simulink model "s_c_nbe_m32k"  (R2018a)
settings: Solver=VariableStepDiscrete  StartTime=0.0  StopTime=1000  RelTol=1e-3
undefined symbols (not defined in the file): fft_stages, n_taps, output_bits, pfb_coeff_gen_calc, xengbits
libraries: xbsIndex_r4 x23714, casper_library_misc x17, xps_library x4, casper_library_scopes x4, xbsReplacements_r4 x4
(part 155 of 171)

== system s_c_nbe_m32k/nb_pfb/pfb_fir_generic2/pfb_fir_taps/bus_adder_tree/add_tree1 ==
  sync : Inport
  din1 : Inport  Port=2
  din2 : Inport  Port=3
  din3 : Inport  Port=4
  din4 : Inport  Port=5
  addr1 : xbsIndex_r4/AddSub  mode=Addition  use_carryin=off  use_carryout=off  en=off  latency=7  precision=Full  arith_type=Unsigned  n_bits=16  bin_pt=14  quantization=Truncate  overflow=Wrap  use_behavioral_HDL=on  hw_selection=Fabric  pipelined=on  use_rpm=on  dbl_ovrd=off  block_type=addsub
  addr2 : xbsIndex_r4/AddSub  mode=Addition  use_carryin=off  use_carryout=off  en=off  latency=7  precision=Full  arith_type=Unsigned  n_bits=16  bin_pt=14  quantization=Truncate  overflow=Wrap  use_behavioral_HDL=on  hw_selection=Fabric  pipelined=on  use_rpm=on  dbl_ovrd=off  block_type=addsub
  addr3 : xbsIndex_r4/AddSub  mode=Addition  use_carryin=off  use_carryout=off  en=off  latency=7  precision=Full  arith_type=Unsigned  n_bits=16  bin_pt=14  quantization=Truncate  overflow=Wrap  use_behavioral_HDL=on  hw_selection=Fabric  pipelined=on  use_rpm=on  dbl_ovrd=off  block_type=addsub
  sync_delay : xbsIndex_r4/Delay  rst=off  infoeditControl=Selection of Reset will increase slice count due to use of real FFs and instead of SRLs  en=off  latency=14  reg_retiming=on  dbl_ovrd=off  block_type=delay
      settings: block_version=11.4
  sync_out : Outport
  dout : Outport  Port=2
  wires:
  addr3/1 -> dout/1
  addr2/1 -> addr3/2
  addr1/1 -> addr3/1
  din4/1 -> addr2/2
  din3/1 -> addr2/1
  din2/1 -> addr1/2
  din1/1 -> addr1/1
  sync_delay/1 -> sync_out/1
  sync/1 -> sync_delay/1

== system s_c_nbe_m32k/nb_pfb/pfb_fir_generic2/pfb_fir_taps/bus_adder_tree/d_bussify ==
  in1 : Inport
  in2 : Inport  Port=2
  concatenate : xbsIndex_r4/Concat  num_inputs=2  dbl_ovrd=off  block_type=concat
  reinterpret1 : xbsIndex_r4/Reinterpret  force_arith_type=on  arith_type=Unsigned  force_bin_pt=on  bin_pt=0  block_type=reinterpret
      settings: infoedit="Changes signal type without altering the binary representation.   You can changed the signal between signed and unsigned, and relocate the binary point.<br><br>Hardware notes: In hardware this block costs nothing.<br><br>Example:  Suppose the input is 6 bits wide, signed, with 2 fractional bits, and the output is forced to unsigned with 0 fractional bits.  Then an input of -2.0 (1110.00 in binary 2's complement) becomes an output of 56 (111000 in binary)."
  reinterpret2 : xbsIndex_r4/Reinterpret  force_arith_type=on  arith_type=Unsigned  force_bin_pt=on  bin_pt=0  block_type=reinterpret
      settings: infoedit="Changes signal type without altering the binary representation.   You can changed the signal between signed and unsigned, and relocate the binary point.<br><br>Hardware notes: In hardware this block costs nothing.<br><br>Example:  Suppose the input is 6 bits wide, signed, with 2 fractional bits, and the output is forced to unsigned with 0 fractional bits.  Then an input of -2.0 (1110.00 in binary 2's complement) becomes an output of 56 (111000 in binary)."
  bus_out : Outport
  wires:
  reinterpret2/1 -> concatenate/2
  in2/1 -> reinterpret2/1
  reinterpret1/1 -> concatenate/1
  in1/1 -> reinterpret1/1
  concatenate/1 -> bus_out/1

== system s_c_nbe_m32k/nb_pfb/pfb_fir_generic2/pfb_fir_taps/bus_adder_tree/expand0 ==
  bus_in : Inport
  reinterpret1 : xbsIndex_r4/Reinterpret  force_arith_type=on  arith_type="Signed  (2's comp)"  force_bin_pt=on  bin_pt=34  block_type=reinterpret
  reinterpret2 : xbsIndex_r4/Reinterpret  force_arith_type=on  arith_type="Signed  (2's comp)"  force_bin_pt=on  bin_pt=34  block_type=reinterpret
  slice1 : xbsIndex_r4/Slice  nbits=36  boolean_output=off  mode=Upper Bit Location + Width  bit1=-36  base1=MSB of Input  bit0=0  base0=LSB of Input  dbl_ovrd=off  block_type=slice
  slice2 : xbsIndex_r4/Slice  nbits=36  boolean_output=off  mode=Upper Bit Location + Width  bit1=0  base1=MSB of Input  bit0=0  base0=LSB of Input  dbl_ovrd=off  block_type=slice
  msb_out2 : Outport
  lsb_out1 : Outport  Port=2
  wires:
  bus_in/1 -> slice2/1, slice1/1
  slice2/1 -> reinterpret2/1
  reinterpret2/1 -> msb_out2/1
  slice1/1 -> reinterpret1/1
  reinterpret1/1 -> lsb_out1/1

== system s_c_nbe_m32k/nb_pfb/pfb_fir_generic2/pfb_fir_taps/bus_adder_tree/expand1 ==
  bus_in : Inport
  reinterpret1 : xbsIndex_r4/Reinterpret  force_arith_type=on  arith_type="Signed  (2's comp)"  force_bin_pt=on  bin_pt=34  block_type=reinterpret
  reinterpret2 : xbsIndex_r4/Reinterpret  force_arith_type=on  arith_type="Signed  (2's comp)"  force_bin_pt=on  bin_pt=34  block_type=reinterpret
  slice1 : xbsIndex_r4/Slice  nbits=36  boolean_output=off  mode=Upper Bit Location + Width  bit1=-36  base1=MSB of Input  bit0=0  base0=LSB of Input  dbl_ovrd=off  block_type=slice
  slice2 : xbsIndex_r4/Slice  nbits=36  boolean_output=off  mode=Upper Bit Location + Width  bit1=0  base1=MSB of Input  bit0=0  base0=LSB of Input  dbl_ovrd=off  block_type=slice
  msb_out2 : Outport
  lsb_out1 : Outport  Port=2
  wires:
  bus_in/1 -> slice2/1, slice1/1
  slice2/1 -> reinterpret2/1
  reinterpret2/1 -> msb_out2/1
  slice1/1 -> reinterpret1/1
  reinterpret1/1 -> lsb_out1/1

== system s_c_nbe_m32k/nb_pfb/pfb_fir_generic2/pfb_fir_taps/bus_adder_tree/expand2 ==
  bus_in : Inport
  reinterpret1 : xbsIndex_r4/Reinterpret  force_arith_type=on  arith_type="Signed  (2's comp)"  force_bin_pt=on  bin_pt=34  block_type=reinterpret
  reinterpret2 : xbsIndex_r4/Reinterpret  force_arith_type=on  arith_type="Signed  (2's comp)"  force_bin_pt=on  bin_pt=34  block_type=reinterpret
  slice1 : xbsIndex_r4/Slice  nbits=36  boolean_output=off  mode=Upper Bit Location + Width  bit1=-36  base1=MSB of Input  bit0=0  base0=LSB of Input  dbl_ovrd=off  block_type=slice
  slice2 : xbsIndex_r4/Slice  nbits=36  boolean_output=off  mode=Upper Bit Location + Width  bit1=0  base1=MSB of Input  bit0=0  base0=LSB of Input  dbl_ovrd=off  block_type=slice
  msb_out2 : Outport
  lsb_out1 : Outport  Port=2
  wires:
  bus_in/1 -> slice2/1, slice1/1
  slice2/1 -> reinterpret2/1
  reinterpret2/1 -> msb_out2/1
  slice1/1 -> reinterpret1/1
  reinterpret1/1 -> lsb_out1/1

== system s_c_nbe_m32k/nb_pfb/pfb_fir_generic2/pfb_fir_taps/bus_adder_tree/expand3 ==
  bus_in : Inport
  reinterpret1 : xbsIndex_r4/Reinterpret  force_arith_type=on  arith_type="Signed  (2's comp)"  force_bin_pt=on  bin_pt=34  block_type=reinterpret
  reinterpret2 : xbsIndex_r4/Reinterpret  force_arith_type=on  arith_type="Signed  (2's comp)"  force_bin_pt=on  bin_pt=34  block_type=reinterpret
  slice1 : xbsIndex_r4/Slice  nbits=36  boolean_output=off  mode=Upper Bit Location + Width  bit1=-36  base1=MSB of Input  bit0=0  base0=LSB of Input  dbl_ovrd=off  block_type=slice
  slice2 : xbsIndex_r4/Slice  nbits=36  boolean_output=off  mode=Upper Bit Location + Width  bit1=0  base1=MSB of Input  bit0=0  base0=LSB of Input  dbl_ovrd=off  block_type=slice
  msb_out2 : Outport
  lsb_out1 : Outport  Port=2
  wires:
  bus_in/1 -> slice2/1, slice1/1
  slice2/1 -> reinterpret2/1
  reinterpret2/1 -> msb_out2/1
  slice1/1 -> reinterpret1/1
  reinterpret1/1 -> lsb_out1/1

== system s_c_nbe_m32k/nb_pfb/pfb_fir_generic2/pfb_fir_taps/bus_mult/a*b_bussify ==
  in1 : Inport
  in2 : Inport  Port=2
  in3 : Inport  Port=3
  in4 : Inport  Port=4
  in5 : Inport  Port=5
  in6 : Inport  Port=6
  in7 : Inport  Port=7
  in8 : Inport  Port=8
  concatenate : xbsIndex_r4/Concat  num_inputs=8  dbl_ovrd=off  block_type=concat
  reinterpret{1..8} (8 alike) : xbsIndex_r4/Reinterpret  force_arith_type=on  arith_type=Unsigned  force_bin_pt=on  bin_pt=0  block_type=reinterpret
      reinterpret1 settings: infoedit="Changes signal type without altering the binary representation.   You can changed the signal between signed and unsigned, and relocate the binary point.<br><br>Hardware notes: In hardware this block costs nothing.<br><br>Example:  Suppose the input is 6 bits wide, signed, with 2 fractional bits, and the output is forced to unsigned with 0 fractional bits.  Then an input of -2.0 (1110.00 in binary 2's complement) becomes an output of 56 (111000 in binary)."
      reinterpret2 settings: infoedit="Changes signal type without altering the binary representation.   You can changed the signal between signed and unsigned, and relocate the binary point.<br><br>Hardware notes: In hardware this block costs nothing.<br><br>Example:  Suppose the input is 6 bits wide, signed, with 2 fractional bits, and the output is forced to unsigned with 0 fractional bits.  Then an input of -2.0 (1110.00 in binary 2's complement) becomes an output of 56 (111000 in binary)."
  bus_out : Outport
  wires:
  reinterpret8/1 -> concatenate/8
  in8/1 -> reinterpret8/1
  reinterpret7/1 -> concatenate/7
  in7/1 -> reinterpret7/1
  reinterpret6/1 -> concatenate/6
  in6/1 -> reinterpret6/1
  reinterpret5/1 -> concatenate/5
  in5/1 -> reinterpret5/1
  reinterpret4/1 -> concatenate/4
  in4/1 -> reinterpret4/1
  reinterpret3/1 -> concatenate/3
  in3/1 -> reinterpret3/1
  reinterpret2/1 -> concatenate/2
  in2/1 -> reinterpret2/1
  reinterpret1/1 -> concatenate/1
  in1/1 -> reinterpret1/1
  concatenate/1 -> bus_out/1

== system s_c_nbe_m32k/nb_pfb/pfb_fir_generic2/pfb_fir_taps/bus_mult/a_debus ==
  bus_in : Inport
  reinterpret{1..8} (8 alike) : xbsIndex_r4/Reinterpret  force_arith_type=on  arith_type="Signed  (2's comp)"  force_bin_pt=on  bin_pt=17  block_type=reinterpret
  slice1 : xbsIndex_r4/Slice  nbits=18  boolean_output=off  mode=Upper Bit Location + Width  bit1=-126  base1=MSB of Input  bit0=0  base0=LSB of Input  dbl_ovrd=off  block_type=slice
  slice2 : xbsIndex_r4/Slice  nbits=18  boolean_output=off  mode=Upper Bit Location + Width  bit1=-108  base1=MSB of Input  bit0=0  base0=LSB of Input  dbl_ovrd=off  block_type=slice
  slice3 : xbsIndex_r4/Slice  nbits=18  boolean_output=off  mode=Upper Bit Location + Width  bit1=-90  base1=MSB of Input  bit0=0  base0=LSB of Input  dbl_ovrd=off  block_type=slice
  slice4 : xbsIndex_r4/Slice  nbits=18  boolean_output=off  mode=Upper Bit Location + Width  bit1=-72  base1=MSB of Input  bit0=0  base0=LSB of Input  dbl_ovrd=off  block_type=slice
  slice5 : xbsIndex_r4/Slice  nbits=18  boolean_output=off  mode=Upper Bit Location + Width  bit1=-54  base1=MSB of Input  bit0=0  base0=LSB of Input  dbl_ovrd=off  block_type=slice
  slice6 : xbsIndex_r4/Slice  nbits=18  boolean_output=off  mode=Upper Bit Location + Width  bit1=-36  base1=MSB of Input  bit0=0  base0=LSB of Input  dbl_ovrd=off  block_type=slice
  slice7 : xbsIndex_r4/Slice  nbits=18  boolean_output=off  mode=Upper Bit Location + Width  bit1=-18  base1=MSB of Input  bit0=0  base0=LSB of Input  dbl_ovrd=off  block_type=slice
  slice8 : xbsIndex_r4/Slice  nbits=18  boolean_output=off  mode=Upper Bit Location + Width  bit1=0  base1=MSB of Input  bit0=0  base0=LSB of Input  dbl_ovrd=off  block_type=slice
  msb_out8 : Outport
  out7 : Outport  Port=2
  out6 : Outport  Port=3
  out5 : Outport  Port=4
  out4 : Outport  Port=5
  out3 : Outport  Port=6
  out2 : Outport  Port=7
  lsb_out1 : Outport  Port=8
  wires:
  bus_in/1 -> slice8/1, slice7/1, slice6/1, slice5/1, slice4/1, slice3/1, slice2/1, slice1/1
  slice8/1 -> reinterpret8/1
  reinterpret8/1 -> msb_out8/1
  slice7/1 -> reinterpret7/1
  reinterpret7/1 -> out7/1
  slice6/1 -> reinterpret6/1
  reinterpret6/1 -> out6/1
  slice5/1 -> reinterpret5/1
  reinterpret5/1 -> out5/1
  slice4/1 -> reinterpret4/1
  reinterpret4/1 -> out4/1
  slice3/1 -> reinterpret3/1
  reinterpret3/1 -> out3/1
  slice2/1 -> reinterpret2/1
  reinterpret2/1 -> out2/1
  slice1/1 -> reinterpret1/1
  reinterpret1/1 -> lsb_out1/1

== system s_c_nbe_m32k/nb_pfb/pfb_fir_generic2/pfb_fir_taps/bus_mult/b_debus ==
  bus_in : Inport
  reinterpret{1..8} (8 alike) : xbsIndex_r4/Reinterpret  force_arith_type=on  arith_type="Signed  (2's comp)"  force_bin_pt=on  bin_pt=17  block_type=reinterpret
  slice1 : xbsIndex_r4/Slice  nbits=18  boolean_output=off  mode=Upper Bit Location + Width  bit1=-126  base1=MSB of Input  bit0=0  base0=LSB of Input  dbl_ovrd=off  block_type=slice
  slice2 : xbsIndex_r4/Slice  nbits=18  boolean_output=off  mode=Upper Bit Location + Width  bit1=-108  base1=MSB of Input  bit0=0  base0=LSB of Input  dbl_ovrd=off  block_type=slice
  slice3 : xbsIndex_r4/Slice  nbits=18  boolean_output=off  mode=Upper Bit Location + Width  bit1=-90  base1=MSB of Input  bit0=0  base0=LSB of Input  dbl_ovrd=off  block_type=slice
  slice4 : xbsIndex_r4/Slice  nbits=18  boolean_output=off  mode=Upper Bit Location + Width  bit1=-72  base1=MSB of Input  bit0=0  base0=LSB of Input  dbl_ovrd=off  block_type=slice
  slice5 : xbsIndex_r4/Slice  nbits=18  boolean_output=off  mode=Upper Bit Location + Width  bit1=-54  base1=MSB of Input  bit0=0  base0=LSB of Input  dbl_ovrd=off  block_type=slice
  slice6 : xbsIndex_r4/Slice  nbits=18  boolean_output=off  mode=Upper Bit Location + Width  bit1=-36  base1=MSB of Input  bit0=0  base0=LSB of Input  dbl_ovrd=off  block_type=slice
  slice7 : xbsIndex_r4/Slice  nbits=18  boolean_output=off  mode=Upper Bit Location + Width  bit1=-18  base1=MSB of Input  bit0=0  base0=LSB of Input  dbl_ovrd=off  block_type=slice
  slice8 : xbsIndex_r4/Slice  nbits=18  boolean_output=off  mode=Upper Bit Location + Width  bit1=0  base1=MSB of Input  bit0=0  base0=LSB of Input  dbl_ovrd=off  block_type=slice
  msb_out8 : Outport
  out7 : Outport  Port=2
  out6 : Outport  Port=3
  out5 : Outport  Port=4
  out4 : Outport  Port=5
  out3 : Outport  Port=6
  out2 : Outport  Port=7
  lsb_out1 : Outport  Port=8
  wires:
  bus_in/1 -> slice8/1, slice7/1, slice6/1, slice5/1, slice4/1, slice3/1, slice2/1, slice1/1
  slice8/1 -> reinterpret8/1
  reinterpret8/1 -> msb_out8/1
  slice7/1 -> reinterpret7/1
  reinterpret7/1 -> out7/1
  slice6/1 -> reinterpret6/1
  reinterpret6/1 -> out6/1
  slice5/1 -> reinterpret5/1
  reinterpret5/1 -> out5/1
  slice4/1 -> reinterpret4/1
  reinterpret4/1 -> out4/1
  slice3/1 -> reinterpret3/1
  reinterpret3/1 -> out3/1
  slice2/1 -> reinterpret2/1
  reinterpret2/1 -> out2/1
  slice1/1 -> reinterpret1/1
  reinterpret1/1 -> lsb_out1/1

== system s_c_nbe_m32k/nb_pfb/pfb_fir_generic2/pfb_fir_taps/bus_mult/repa ==
  in : Inport
  bussify : Subsystem  mask(bus_create){inputNum=1}
      mask prompts: inputNum "Number of inputs:"
      mask init:
      | bus_create_init(gcb,...
      |     'inputNum', inputNum);
  out : Outport
  wires:
  bussify/1(bus_out) -> out/1
  in/1 -> bussify/1(in1)

== system s_c_nbe_m32k/nb_pfb/pfb_fir_generic2/pfb_fir_taps/bus_mult/repb ==
  in : Inport
  bussify : Subsystem  mask(bus_create){inputNum=1}
      mask prompts: inputNum "Number of inputs:"
      mask init:
      | bus_create_init(gcb,...
      |     'inputNum', inputNum);
  out : Outport
  wires:
  bussify/1(bus_out) -> out/1
  in/1 -> bussify/1(in1)

== system s_c_nbe_m32k/nb_pfb/pfb_fir_generic2/pfb_fir_taps/tap_delays/A_bussify0 ==
  in1 : Inport
  in2 : Inport  Port=2
  in3 : Inport  Port=3
  in4 : Inport  Port=4
  in5 : Inport  Port=5
  in6 : Inport  Port=6
  in7 : Inport  Port=7
  in8 : Inport  Port=8
  in9 : Inport  Port=9
  in10 : Inport  Port=10
  in11 : Inport  Port=11
  in12 : Inport  Port=12
  in13 : Inport  Port=13
  in14 : Inport  Port=14
  in15 : Inport  Port=15
  in16 : Inport  Port=16
  in17 : Inport  Port=17
  in18 : Inport  Port=18
  in19 : Inport  Port=19
  in20 : Inport  Port=20
  in21 : Inport  Port=21
  in22 : Inport  Port=22
  in23 : Inport  Port=23
  in24 : Inport  Port=24
  in25 : Inport  Port=25
  in26 : Inport  Port=26
  in27 : Inport  Port=27
  in28 : Inport  Port=28
  in29 : Inport  Port=29
  in30 : Inport  Port=30
  in31 : Inport  Port=31
  in32 : Inport  Port=32
  in33 : Inport  Port=33
  in34 : Inport  Port=34
  in35 : Inport  Port=35
  in36 : Inport  Port=36
  in37 : Inport  Port=37
  in38 : Inport  Port=38
  in39 : Inport  Port=39
  in40 : Inport  Port=40
  in41 : Inport  Port=41
  in42 : Inport  Port=42
  in43 : Inport  Port=43
  in44 : Inport  Port=44
  in45 : Inport  Port=45
  in46 : Inport  Port=46
  in47 : Inport  Port=47
  in48 : Inport  Port=48
  in49 : Inport  Port=49
  in50 : Inport  Port=50
  in51 : Inport  Port=51
  in52 : Inport  Port=52
  in53 : Inport  Port=53
  in54 : Inport  Port=54
  in55 : Inport  Port=55
  in56 : Inport  Port=56
  in57 : Inport  Port=57
  in58 : Inport  Port=58
  in59 : Inport  Port=59
  in60 : Inport  Port=60
  in61 : Inport  Port=61
  in62 : Inport  Port=62
  in63 : Inport  Port=63
  in64 : Inport  Port=64
  in65 : Inport  Port=65
  in66 : Inport  Port=66
  in67 : Inport  Port=67
  in68 : Inport  Port=68
  in69 : Inport  Port=69
  in70 : Inport  Port=70
  in71 : Inport  Port=71
  in72 : Inport  Port=72
  in73 : Inport  Port=73
  in74 : Inport  Port=74
  in75 : Inport  Port=75
  in76 : Inport  Port=76
  in77 : Inport  Port=77
  in78 : Inport  Port=78
  in79 : Inport  Port=79
  in80 : Inport  Port=80
  in81 : Inport  Port=81
  in82 : Inport  Port=82
  in83 : Inport  Port=83
  in84 : Inport  Port=84
  in85 : Inport  Port=85
  in86 : Inport  Port=86
  in87 : Inport  Port=87
  in88 : Inport  Port=88
  in89 : Inport  Port=89
  in90 : Inport  Port=90
  in91 : Inport  Port=91
  in92 : Inport  Port=92
  in93 : Inport  Port=93
  in94 : Inport  Port=94
  in95 : Inport  Port=95
  in96 : Inport  Port=96
  in97 : Inport  Port=97
  in98 : Inport  Port=98
  in99 : Inport  Port=99
  in100 : Inport  Port=100
  in101 : Inport  Port=101
  in102 : Inport  Port=102
  in103 : Inport  Port=103
  in104 : Inport  Port=104
  in105 : Inport  Port=105
  in106 : Inport  Port=106
  in107 : Inport  Port=107
  in108 : Inport  Port=108
  concatenate : xbsIndex_r4/Concat  num_inputs=108  dbl_ovrd=off  block_type=concat
  reinterpret{1..108} (108 alike) : xbsIndex_r4/Reinterpret  force_arith_type=on  arith_type=Unsigned  force_bin_pt=on  bin_pt=0  block_type=reinterpret
      reinterpret1 settings: infoedit="Changes signal type without altering the binary representation.   You can changed the signal between signed and unsigned, and relocate the binary point.<br><br>Hardware notes: In hardware this block costs nothing.<br><br>Example:  Suppose the input is 6 bits wide, signed, with 2 fractional bits, and the output is forced to unsigned with 0 fractional bits.  Then an input of -2.0 (1110.00 in binary 2's complement) becomes an output of 56 (111000 in binary)."
      reinterpret2 settings: infoedit="Changes signal type without altering the binary representation.   You can changed the signal between signed and unsigned, and relocate the binary point.<br><br>Hardware notes: In hardware this block costs nothing.<br><br>Example:  Suppose the input is 6 bits wide, signed, with 2 fractional bits, and the output is forced to unsigned with 0 fractional bits.  Then an input of -2.0 (1110.00 in binary 2's complement) becomes an output of 56 (111000 in binary)."
  bus_out : Outport
  wires:
  reinterpret108/1 -> concatenate/108
  in108/1 -> reinterpret108/1
  reinterpret107/1 -> concatenate/107
  in107/1 -> reinterpret107/1
  reinterpret106/1 -> concatenate/106
  in106/1 -> reinterpret106/1
  reinterpret105/1 -> concatenate/105
  in105/1 -> reinterpret105/1
  reinterpret104/1 -> concatenate/104
  in104/1 -> reinterpret104/1
  reinterpret103/1 -> concatenate/103
  in103/1 -> reinterpret103/1
  reinterpret102/1 -> concatenate/102
  in102/1 -> reinterpret102/1
  reinterpret101/1 -> concatenate/101
  in101/1 -> reinterpret101/1
  reinterpret100/1 -> concatenate/100
  in100/1 -> reinterpret100/1
  reinterpret99/1 -> concatenate/99
  in99/1 -> reinterpret99/1
  reinterpret98/1 -> concatenate/98
  in98/1 -> reinterpret98/1
  reinterpret97/1 -> concatenate/97
  in97/1 -> reinterpret97/1
  reinterpret96/1 -> concatenate/96
  in96/1 -> reinterpret96/1
  reinterpret95/1 -> concatenate/95
  in95/1 -> reinterpret95/1
  reinterpret94/1 -> concatenate/94
  in94/1 -> reinterpret94/1
  reinterpret93/1 -> concatenate/93
  in93/1 -> reinterpret93/1
  reinterpret92/1 -> concatenate/92
  in92/1 -> reinterpret92/1
  reinterpret91/1 -> concatenate/91
  in91/1 -> reinterpret91/1
  reinterpret90/1 -> concatenate/90
  in90/1 -> reinterpret90/1
  reinterpret89/1 -> concatenate/89
  in89/1 -> reinterpret89/1
  reinterpret88/1 -> concatenate/88
  in88/1 -> reinterpret88/1
  reinterpret87/1 -> concatenate/87
  in87/1 -> reinterpret87/1
  reinterpret86/1 -> concatenate/86
  in86/1 -> reinterpret86/1
  reinterpret85/1 -> concatenate/85
  in85/1 -> reinterpret85/1
  reinterpret84/1 -> concatenate/84
  in84/1 -> reinterpret84/1
  reinterpret83/1 -> concatenate/83
  in83/1 -> reinterpret83/1
  reinterpret82/1 -> concatenate/82
  in82/1 -> reinterpret82/1
  reinterpret81/1 -> concatenate/81
  in81/1 -> reinterpret81/1
  reinterpret80/1 -> concatenate/80
  in80/1 -> reinterpret80/1
  reinterpret79/1 -> concatenate/79
  in79/1 -> reinterpret79/1
  reinterpret78/1 -> concatenate/78
  in78/1 -> reinterpret78/1
  reinterpret77/1 -> concatenate/77
  in77/1 -> reinterpret77/1
  reinterpret76/1 -> concatenate/76
  in76/1 -> reinterpret76/1
  reinterpret75/1 -> concatenate/75
  in75/1 -> reinterpret75/1
  reinterpret74/1 -> concatenate/74
  in74/1 -> reinterpret74/1
  reinterpret73/1 -> concatenate/73
  in73/1 -> reinterpret73/1
  reinterpret72/1 -> concatenate/72
  in72/1 -> reinterpret72/1
  reinterpret71/1 -> concatenate/71
  in71/1 -> reinterpret71/1
  reinterpret70/1 -> concatenate/70
  in70/1 -> reinterpret70/1
  reinterpret69/1 -> concatenate/69
  in69/1 -> reinterpret69/1
  reinterpret68/1 -> concatenate/68
  in68/1 -> reinterpret68/1
  reinterpret67/1 -> concatenate/67
  in67/1 -> reinterpret67/1
  reinterpret66/1 -> concatenate/66
  in66/1 -> reinterpret66/1
  reinterpret65/1 -> concatenate/65
  in65/1 -> reinterpret65/1
  reinterpret64/1 -> concatenate/64
  in64/1 -> reinterpret64/1
  reinterpret63/1 -> concatenate/63
  in63/1 -> reinterpret63/1
  reinterpret62/1 -> concatenate/62
  in62/1 -> reinterpret62/1
  reinterpret61/1 -> concatenate/61
  in61/1 -> reinterpret61/1
  reinterpret60/1 -> concatenate/60
  in60/1 -> reinterpret60/1
  reinterpret59/1 -> concatenate/59
  in59/1 -> reinterpret59/1
  reinterpret58/1 -> concatenate/58
  in58/1 -> reinterpret58/1
  reinterpret57/1 -> concatenate/57
  in57/1 -> reinterpret57/1
  reinterpret56/1 -> concatenate/56
  in56/1 -> reinterpret56/1
  reinterpret55/1 -> concatenate/55
  in55/1 -> reinterpret55/1
  reinterpret54/1 -> concatenate/54
  in54/1 -> reinterpret54/1
  reinterpret53/1 -> concatenate/53
  in53/1 -> reinterpret53/1
  reinterpret52/1 -> concatenate/52
  in52/1 -> reinterpret52/1
  reinterpret51/1 -> concatenate/51
  in51/1 -> reinterpret51/1
  reinterpret50/1 -> concatenate/50
  in50/1 -> reinterpret50/1
  reinterpret49/1 -> concatenate/49
  in49/1 -> reinterpret49/1
  reinterpret48/1 -> concatenate/48
  in48/1 -> reinterpret48/1
  reinterpret47/1 -> concatenate/47
  in47/1 -> reinterpret47/1
  reinterpret46/1 -> concatenate/46
  in46/1 -> reinterpret46/1
  reinterpret45/1 -> concatenate/45
  in45/1 -> reinterpret45/1
  reinterpret44/1 -> concatenate/44
  in44/1 -> reinterpret44/1
  reinterpret43/1 -> concatenate/43
  in43/1 -> reinterpret43/1
  reinterpret42/1 -> concatenate/42
  in42/1 -> reinterpret42/1
  reinterpret41/1 -> concatenate/41
  in41/1 -> reinterpret41/1
  reinterpret40/1 -> concatenate/40
  in40/1 -> reinterpret40/1
  reinterpret39/1 -> concatenate/39
  in39/1 -> reinterpret39/1
  reinterpret38/1 -> concatenate/38
  in38/1 -> reinterpret38/1
  reinterpret37/1 -> concatenate/37
  in37/1 -> reinterpret37/1
  reinterpret36/1 -> concatenate/36
  in36/1 -> reinterpret36/1
  reinterpret35/1 -> concatenate/35
  in35/1 -> reinterpret35/1
  reinterpret34/1 -> concatenate/34
  in34/1 -> reinterpret34/1
  reinterpret33/1 -> concatenate/33
  in33/1 -> reinterpret33/1
  reinterpret32/1 -> concatenate/32
  in32/1 -> reinterpret32/1
  reinterpret31/1 -> concatenate/31
  in31/1 -> reinterpret31/1
  reinterpret30/1 -> concatenate/30
  in30/1 -> reinterpret30/1
  reinterpret29/1 -> concatenate/29
  in29/1 -> reinterpret29/1
  reinterpret28/1 -> concatenate/28
  in28/1 -> reinterpret28/1
  reinterpret27/1 -> concatenate/27
  in27/1 -> reinterpret27/1
  reinterpret26/1 -> concatenate/26
  in26/1 -> reinterpret26/1
  reinterpret25/1 -> concatenate/25
  in25/1 -> reinterpret25/1
  reinterpret24/1 -> concatenate/24
  in24/1 -> reinterpret24/1
  reinterpret23/1 -> concatenate/23
  in23/1 -> reinterpret23/1
  reinterpret22/1 -> concatenate/22
  in22/1 -> reinterpret22/1
  reinterpret21/1 -> concatenate/21
  in21/1 -> reinterpret21/1
  reinterpret20/1 -> concatenate/20
  in20/1 -> reinterpret20/1
  reinterpret19/1 -> concatenate/19
  in19/1 -> reinterpret19/1
  reinterpret18/1 -> concatenate/18
  in18/1 -> reinterpret18/1
  reinterpret17/1 -> concatenate/17
  in17/1 -> reinterpret17/1
  reinterpret16/1 -> concatenate/16
  in16/1 -> reinterpret16/1
  reinterpret15/1 -> concatenate/15
  in15/1 -> reinterpret15/1
  reinterpret14/1 -> concatenate/14
  in14/1 -> reinterpret14/1
  reinterpret13/1 -> concatenate/13
  in13/1 -> reinterpret13/1
  reinterpret12/1 -> concatenate/12
  in12/1 -> reinterpret12/1
  reinterpret11/1 -> concatenate/11
  in11/1 -> reinterpret11/1
  reinterpret10/1 -> concatenate/10
  in10/1 -> reinterpret10/1
  reinterpret9/1 -> concatenate/9
  in9/1 -> reinterpret9/1
  reinterpret8/1 -> concatenate/8
  in8/1 -> reinterpret8/1
  reinterpret7/1 -> concatenate/7
  in7/1 -> reinterpret7/1
  reinterpret6/1 -> concatenate/6
  in6/1 -> reinterpret6/1
  reinterpret5/1 -> concatenate/5
  in5/1 -> reinterpret5/1
  reinterpret4/1 -> concatenate/4
  in4/1 -> reinterpret4/1
  reinterpret3/1 -> concatenate/3
  in3/1 -> reinterpret3/1
  reinterpret2/1 -> concatenate/2
  in2/1 -> reinterpret2/1
  reinterpret1/1 -> concatenate/1
  in1/1 -> reinterpret1/1
  concatenate/1 -> bus_out/1

== system s_c_nbe_m32k/nb_pfb/pfb_fir_generic2/pfb_fir_taps/tap_delays/B_bussify0 ==
  in1 : Inport
  in2 : Inport  Port=2
  in3 : Inport  Port=3
  in4 : Inport  Port=4
  in5 : Inport  Port=5
  in6 : Inport  Port=6
  in7 : Inport  Port=7
  in8 : Inport  Port=8
  in9 : Inport  Port=9
  in10 : Inport  Port=10
  in11 : Inport  Port=11
  in12 : Inport  Port=12
  in13 : Inport  Port=13
  in14 : Inport  Port=14
  in15 : Inport  Port=15
  in16 : Inport  Port=16
  in17 : Inport  Port=17
  in18 : Inport  Port=18
  in19 : Inport  Port=19
  in20 : Inport  Port=20
  in21 : Inport  Port=21
  in22 : Inport  Port=22
  in23 : Inport  Port=23
  in24 : Inport  Port=24
  in25 : Inport  Port=25
  in26 : Inport  Port=26
  in27 : Inport  Port=27
  in28 : Inport  Port=28
  in29 : Inport  Port=29
  in30 : Inport  Port=30
  in31 : Inport  Port=31
  in32 : Inport  Port=32
  in33 : Inport  Port=33
  in34 : Inport  Port=34
  in35 : Inport  Port=35
  in36 : Inport  Port=36
  in37 : Inport  Port=37
  in38 : Inport  Port=38
  in39 : Inport  Port=39
  in40 : Inport  Port=40
  in41 : Inport  Port=41
  in42 : Inport  Port=42
  in43 : Inport  Port=43
  in44 : Inport  Port=44
  in45 : Inport  Port=45
  in46 : Inport  Port=46
  in47 : Inport  Port=47
  in48 : Inport  Port=48
  in49 : Inport  Port=49
  in50 : Inport  Port=50
  in51 : Inport  Port=51
  in52 : Inport  Port=52
  in53 : Inport  Port=53
  in54 : Inport  Port=54
  in55 : Inport  Port=55
  in56 : Inport  Port=56
  in57 : Inport  Port=57
  in58 : Inport  Port=58
  in59 : Inport  Port=59
  in60 : Inport  Port=60
  in61 : Inport  Port=61
  in62 : Inport  Port=62
  in63 : Inport  Port=63
  in64 : Inport  Port=64
  in65 : Inport  Port=65
  in66 : Inport  Port=66
  in67 : Inport  Port=67
  in68 : Inport  Port=68
  in69 : Inport  Port=69
  in70 : Inport  Port=70
  in71 : Inport  Port=71
  in72 : Inport  Port=72
  in73 : Inport  Port=73
  in74 : Inport  Port=74
  in75 : Inport  Port=75
  in76 : Inport  Port=76
  in77 : Inport  Port=77
  in78 : Inport  Port=78
  in79 : Inport  Port=79
  in80 : Inport  Port=80
  in81 : Inport  Port=81
  in82 : Inport  Port=82
  in83 : Inport  Port=83
  in84 : Inport  Port=84
  in85 : Inport  Port=85
  in86 : Inport  Port=86
  in87 : Inport  Port=87
  in88 : Inport  Port=88
  in89 : Inport  Port=89
  in90 : Inport  Port=90
  in91 : Inport  Port=91
  in92 : Inport  Port=92
  in93 : Inport  Port=93
  in94 : Inport  Port=94
  in95 : Inport  Port=95
  in96 : Inport  Port=96
  in97 : Inport  Port=97
  in98 : Inport  Port=98
  in99 : Inport  Port=99
  in100 : Inport  Port=100
  in101 : Inport  Port=101
  in102 : Inport  Port=102
  in103 : Inport  Port=103
  in104 : Inport  Port=104
  in105 : Inport  Port=105
  in106 : Inport  Port=106
  in107 : Inport  Port=107
  in108 : Inport  Port=108
  concatenate : xbsIndex_r4/Concat  num_inputs=108  dbl_ovrd=off  block_type=concat
  reinterpret{1..108} (108 alike) : xbsIndex_r4/Reinterpret  force_arith_type=on  arith_type=Unsigned  force_bin_pt=on  bin_pt=0  block_type=reinterpret
      reinterpret1 settings: infoedit="Changes signal type without altering the binary representation.   You can changed the signal between signed and unsigned, and relocate the binary point.<br><br>Hardware notes: In hardware this block costs nothing.<br><br>Example:  Suppose the input is 6 bits wide, signed, with 2 fractional bits, and the output is forced to unsigned with 0 fractional bits.  Then an input of -2.0 (1110.00 in binary 2's complement) becomes an output of 56 (111000 in binary)."
      reinterpret2 settings: infoedit="Changes signal type without altering the binary representation.   You can changed the signal between signed and unsigned, and relocate the binary point.<br><br>Hardware notes: In hardware this block costs nothing.<br><br>Example:  Suppose the input is 6 bits wide, signed, with 2 fractional bits, and the output is forced to unsigned with 0 fractional bits.  Then an input of -2.0 (1110.00 in binary 2's complement) becomes an output of 56 (111000 in binary)."
  bus_out : Outport
  wires:
  reinterpret108/1 -> concatenate/108
  in108/1 -> reinterpret108/1
  reinterpret107/1 -> concatenate/107
  in107/1 -> reinterpret107/1
  reinterpret106/1 -> concatenate/106
  in106/1 -> reinterpret106/1
  reinterpret105/1 -> concatenate/105
  in105/1 -> reinterpret105/1
  reinterpret104/1 -> concatenate/104
  in104/1 -> reinterpret104/1
  reinterpret103/1 -> concatenate/103
  in103/1 -> reinterpret103/1
  reinterpret102/1 -> concatenate/102
  in102/1 -> reinterpret102/1
  reinterpret101/1 -> concatenate/101
  in101/1 -> reinterpret101/1
  reinterpret100/1 -> concatenate/100
  in100/1 -> reinterpret100/1
  reinterpret99/1 -> concatenate/99
  in99/1 -> reinterpret99/1
  reinterpret98/1 -> concatenate/98
  in98/1 -> reinterpret98/1
  reinterpret97/1 -> concatenate/97
  in97/1 -> reinterpret97/1
  reinterpret96/1 -> concatenate/96
  in96/1 -> reinterpret96/1
  reinterpret95/1 -> concatenate/95
  in95/1 -> reinterpret95/1
  reinterpret94/1 -> concatenate/94
  in94/1 -> reinterpret94/1
  reinterpret93/1 -> concatenate/93
  in93/1 -> reinterpret93/1
  reinterpret92/1 -> concatenate/92
  in92/1 -> reinterpret92/1
  reinterpret91/1 -> concatenate/91
  in91/1 -> reinterpret91/1
  reinterpret90/1 -> concatenate/90
  in90/1 -> reinterpret90/1
  reinterpret89/1 -> concatenate/89
  in89/1 -> reinterpret89/1
  reinterpret88/1 -> concatenate/88
  in88/1 -> reinterpret88/1
  reinterpret87/1 -> concatenate/87
  in87/1 -> reinterpret87/1
  reinterpret86/1 -> concatenate/86
  in86/1 -> reinterpret86/1
  reinterpret85/1 -> concatenate/85
  in85/1 -> reinterpret85/1
  reinterpret84/1 -> concatenate/84
  in84/1 -> reinterpret84/1
  reinterpret83/1 -> concatenate/83
  in83/1 -> reinterpret83/1
  reinterpret82/1 -> concatenate/82
  in82/1 -> reinterpret82/1
  reinterpret81/1 -> concatenate/81
  in81/1 -> reinterpret81/1
  reinterpret80/1 -> concatenate/80
  in80/1 -> reinterpret80/1
  reinterpret79/1 -> concatenate/79
  in79/1 -> reinterpret79/1
  reinterpret78/1 -> concatenate/78
  in78/1 -> reinterpret78/1
  reinterpret77/1 -> concatenate/77
  in77/1 -> reinterpret77/1
  reinterpret76/1 -> concatenate/76
  in76/1 -> reinterpret76/1
  reinterpret75/1 -> concatenate/75
  in75/1 -> reinterpret75/1
  reinterpret74/1 -> concatenate/74
  in74/1 -> reinterpret74/1
  reinterpret73/1 -> concatenate/73
  in73/1 -> reinterpret73/1
  reinterpret72/1 -> concatenate/72
  in72/1 -> reinterpret72/1
  reinterpret71/1 -> concatenate/71
  in71/1 -> reinterpret71/1
  reinterpret70/1 -> concatenate/70
  in70/1 -> reinterpret70/1
  reinterpret69/1 -> concatenate/69
  in69/1 -> reinterpret69/1
  reinterpret68/1 -> concatenate/68
  in68/1 -> reinterpret68/1
  reinterpret67/1 -> concatenate/67
  in67/1 -> reinterpret67/1
  reinterpret66/1 -> concatenate/66
  in66/1 -> reinterpret66/1
  reinterpret65/1 -> concatenate/65
  in65/1 -> reinterpret65/1
  reinterpret64/1 -> concatenate/64
  in64/1 -> reinterpret64/1
  reinterpret63/1 -> concatenate/63
  in63/1 -> reinterpret63/1
  reinterpret62/1 -> concatenate/62
  in62/1 -> reinterpret62/1
  reinterpret61/1 -> concatenate/61
  in61/1 -> reinterpret61/1
  reinterpret60/1 -> concatenate/60
  in60/1 -> reinterpret60/1
  reinterpret59/1 -> concatenate/59
  in59/1 -> reinterpret59/1
  reinterpret58/1 -> concatenate/58
  in58/1 -> reinterpret58/1
  reinterpret57/1 -> concatenate/57
  in57/1 -> reinterpret57/1
  reinterpret56/1 -> concatenate/56
  in56/1 -> reinterpret56/1
  reinterpret55/1 -> concatenate/55
  in55/1 -> reinterpret55/1
  reinterpret54/1 -> concatenate/54
  in54/1 -> reinterpret54/1
  reinterpret53/1 -> concatenate/53
  in53/1 -> reinterpret53/1
  reinterpret52/1 -> concatenate/52
  in52/1 -> reinterpret52/1
  reinterpret51/1 -> concatenate/51
  in51/1 -> reinterpret51/1
  reinterpret50/1 -> concatenate/50
  in50/1 -> reinterpret50/1
  reinterpret49/1 -> concatenate/49
  in49/1 -> reinterpret49/1
  reinterpret48/1 -> concatenate/48
  in48/1 -> reinterpret48/1
  reinterpret47/1 -> concatenate/47
  in47/1 -> reinterpret47/1
  reinterpret46/1 -> concatenate/46
  in46/1 -> reinterpret46/1
  reinterpret45/1 -> concatenate/45
  in45/1 -> reinterpret45/1
  reinterpret44/1 -> concatenate/44
  in44/1 -> reinterpret44/1
  reinterpret43/1 -> concatenate/43
  in43/1 -> reinterpret43/1
  reinterpret42/1 -> concatenate/42
  in42/1 -> reinterpret42/1
  reinterpret41/1 -> concatenate/41
  in41/1 -> reinterpret41/1
  reinterpret40/1 -> concatenate/40
  in40/1 -> reinterpret40/1
  reinterpret39/1 -> concatenate/39
  in39/1 -> reinterpret39/1
  reinterpret38/1 -> concatenate/38
  in38/1 -> reinterpret38/1
  reinterpret37/1 -> concatenate/37
  in37/1 -> reinterpret37/1
  reinterpret36/1 -> concatenate/36
  in36/1 -> reinterpret36/1
  reinterpret35/1 -> concatenate/35
  in35/1 -> reinterpret35/1
  reinterpret34/1 -> concatenate/34
  in34/1 -> reinterpret34/1
  reinterpret33/1 -> concatenate/33
  in33/1 -> reinterpret33/1
  reinterpret32/1 -> concatenate/32
  in32/1 -> reinterpret32/1
  reinterpret31/1 -> concatenate/31
  in31/1 -> reinterpret31/1
  reinterpret30/1 -> concatenate/30
  in30/1 -> reinterpret30/1
  reinterpret29/1 -> concatenate/29
  in29/1 -> reinterpret29/1
  reinterpret28/1 -> concatenate/28
  in28/1 -> reinterpret28/1
  reinterpret27/1 -> concatenate/27
  in27/1 -> reinterpret27/1
  reinterpret26/1 -> concatenate/26
  in26/1 -> reinterpret26/1
  reinterpret25/1 -> concatenate/25
  in25/1 -> reinterpret25/1
  reinterpret24/1 -> concatenate/24
  in24/1 -> reinterpret24/1
  reinterpret23/1 -> concatenate/23
  in23/1 -> reinterpret23/1
  reinterpret22/1 -> concatenate/22
  in22/1 -> reinterpret22/1
  reinterpret21/1 -> concatenate/21
  in21/1 -> reinterpret21/1
  reinterpret20/1 -> concatenate/20
  in20/1 -> reinterpret20/1
  reinterpret19/1 -> concatenate/19
  in19/1 -> reinterpret19/1
  reinterpret18/1 -> concatenate/18
  in18/1 -> reinterpret18/1
  reinterpret17/1 -> concatenate/17
  in17/1 -> reinterpret17/1
  reinterpret16/1 -> concatenate/16
  in16/1 -> reinterpret16/1
  reinterpret15/1 -> concatenate/15
  in15/1 -> reinterpret15/1
  reinterpret14/1 -> concatenate/14
  in14/1 -> reinterpret14/1
  reinterpret13/1 -> concatenate/13
  in13/1 -> reinterpret13/1
  reinterpret12/1 -> concatenate/12
  in12/1 -> reinterpret12/1
  reinterpret11/1 -> concatenate/11
  in11/1 -> reinterpret11/1
  reinterpret10/1 -> concatenate/10
  in10/1 -> reinterpret10/1
  reinterpret9/1 -> concatenate/9
  in9/1 -> reinterpret9/1
  reinterpret8/1 -> concatenate/8
  in8/1 -> reinterpret8/1
  reinterpret7/1 -> concatenate/7
  in7/1 -> reinterpret7/1
  reinterpret6/1 -> concatenate/6
  in6/1 -> reinterpret6/1
  reinterpret5/1 -> concatenate/5
  in5/1 -> reinterpret5/1
  reinterpret4/1 -> concatenate/4
  in4/1 -> reinterpret4/1
  reinterpret3/1 -> concatenate/3
  in3/1 -> reinterpret3/1
  reinterpret2/1 -> concatenate/2
  in2/1 -> reinterpret2/1
  reinterpret1/1 -> concatenate/1
  in1/1 -> reinterpret1/1
  concatenate/1 -> bus_out/1
